simulink model "SIM_THREE_TANK_SERVO"  (R2025b)
settings: Solver=ode15s  StartTime=0.0  StopTime=1500  RelTol=1e-3
InitFcn:
  | run("index.m")
StopFcn:
  | data_name = "servo_response";
  | save_name = format_file_name(data_name,true);
  | 
  | % Save output data
  | save(save_name,"out")
values from neighbouring files (symbols this model uses):
  adaptParam = 0.15    [index.m]
  hiddenStates = 0    [index.m]
  model_const = struct()    [index.m]
undefined symbols (not defined in the file or in its folder): sigbuilder_block
libraries: simulink x1
settings Model: Creator=HP  LastModifiedBy=USER PC
settings RTWCC: GPUComputeCapability=3.5
settings GRTTargetCC: ArrayLayout=Row-major

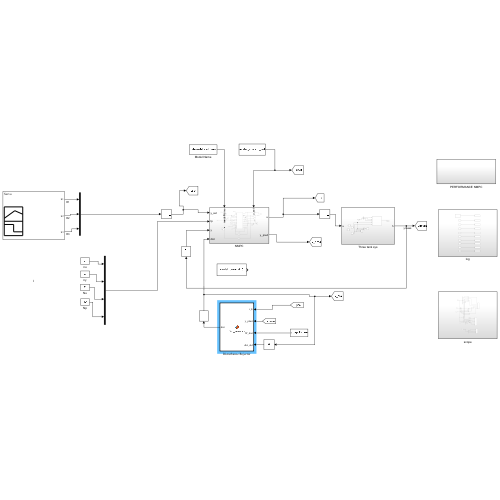
[thumbnail: Simulink's stored preview of the top-level diagram]
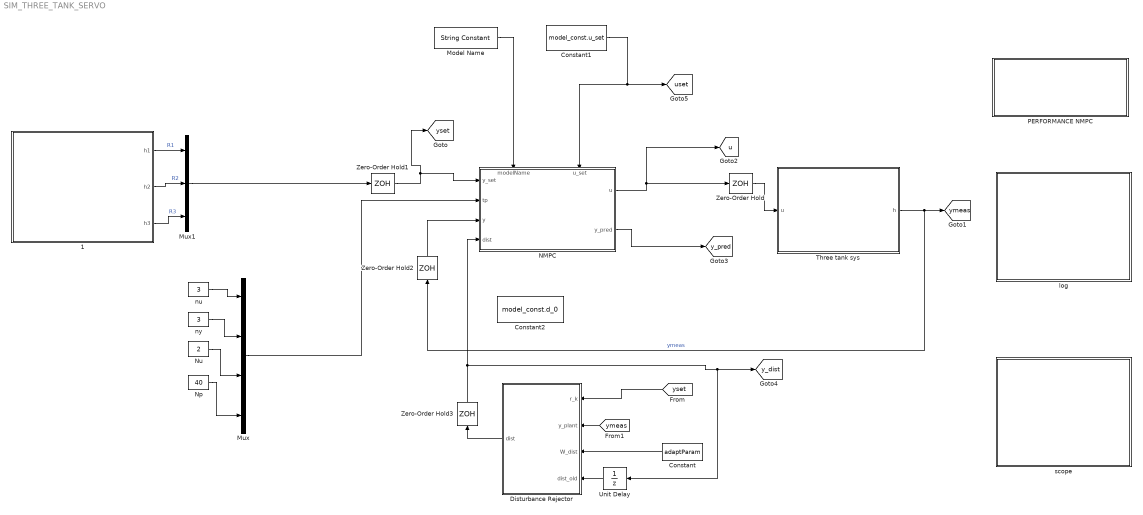
== system SIM_THREE_TANK_SERVO ==
  " 1" : Subsystem  Tag=STV Subsys  LoadFcn=sigbuilder_block('load');  StartFcn=sigbuilder_block('start');  StopFcn=sigbuilder_block('stop');  ClipboardFcn=sigbuilder_block('clipboard');  mask(Sigbuilder block){tuvar=[0:10]}
      mask help: Simulink:masks:SigbuilderBlock_MD
      mask init:
      | if ~strcmp(get_param(bdroot(gcbh),'SimulationStatus'),'stopped') tuvar = sigbuilder_block('maskInit'); end
      settings: CopyFcn=sigbuilder_block('copy');  DeleteFcn=sigbuilder_block('delete');  ModelCloseFcn=sigbuilder_block('modelClose');  PreSaveFcn=sigbuilder_block('preSave');  PauseFcn=sigbuilder_block('pause');  ContinueFcn=sigbuilder_block('continue');  NameChangeFcn=sigbuilder_block('namechange');  OpenFcn=sigbuilder_block('open',[316.5 171.75 805.5 485.25 ]);  CloseFcn=sigbuilder_block('close');
      mask Display: plot(0, 0, 100, 100,[2, 2, 32, 32, 2], [68, 8, 8, 68, 68],[32, 2], [38, 38], [32, 19, 2],[53, 60, 44], [32, 17, 17, 2],[16, 16, 31, 31]);txt = getActiveGroup(gcbh);text(2, 100, txt,'verticalAlignment', 'top');
  Constant : Constant  Value=adaptParam
  Constant1 : Constant  Value=model_const.u_set
  Constant2 : Constant  Value=model_const.d_0  SampleTime=model_const.ts
  Disturbance Rejector : MATLAB Function  TreatAsAtomicUnit=on  SystemSampleTime=10
  Model Name : StringConstant  String=networkModelName
  Mux : Mux
  Mux1 : Mux  Inputs=3
  NMPC : Subsystem
      settings: PortSchema="{\"entries\":[{\"content\":{\"sides\":[{\"content\":{\"connectorIds\":[\"In1\",\"In2\",\"In3\",\"In4\"]},\"type\":\"ConnectorPlacement.EquallySpacedRectSide\",\"uuid\":\"b907109f-bf70-45ef-b014-879f3ccfb12e\"},{\"content\":{\"connectorIds\":[\"Out1\",\"Out2\"],\"side\":\"RIGHT\"},\"type\":\"ConnectorPlacement.EquallySpacedRectSide\",\"uuid\":\"26d01547-fbc3-4b4e-b6e6-c22ae9e5b6d6\"},{\"content\":{\"connectorIds\":[\"In5\",\"In6\"],\"side\":\"TOP\"},\"type\":\"ConnectorPlacement.EquallySpacedRectSide\",\"uuid\":\"f1d5a2c8-1fb2-4706-a136-ec661fe312a9\"},{\"content\":{\"side\":\"BOTTOM\"},\"type\":\"ConnectorPlacement.EquallySpacedRectSide\",\"uuid\":\"24667040-ec86-4e57-b699-830e3f360007\"}]},\"type\":\"ConnectorPlacement.EquallySpacedConnector\",\"uuid\":\"8e79e654-12d3-4871-a9fc-130c68b7f74a\"}],\"packageUris\":[\"http://schema.mathworks.com/mf0/Connector/R2020b\"],\"version\":\"1.0\"}"
  Np : Constant  Value=40
  Nu : Constant  Value=2
  PERFORMANCE NMPC : Subsystem
  Three tank sys : Subsystem
  Unit Delay : UnitDelay  InitialCondition=model_const.d_0  SampleTime=model_const.ts  HasFrameUpgradeWarning=on
  Zero-Order Hold{,1..3} (4 alike) : ZeroOrderHold  SampleTime=model_const.ts
  log : Subsystem
  nu : Constant  Value=3
  ny : Constant  Value=3
  scope : Subsystem
  tag scope: u=global, uset=global, y_dist=global, y_pred=global, ymeas=global, yset=global
  wires:
  Zero-Order Hold1/1 -> NMPC/1(y_set), [yset]
  Nu/1 -> Mux/3
  Constant/1 -> Disturbance Rejector/3(W_dist)
  Unit Delay/1 -> Disturbance Rejector/4(dist_old)
  Mux/1 -> NMPC/2(tp)
  Np/1 -> Mux/4
  [ymeas] -> Disturbance Rejector/2(y_plant)
  NMPC/1(u) -> [u], Zero-Order Hold/1
  Model Name/1 -> NMPC/5(modelName)
  nu/1 -> Mux/1
  ny/1 -> Mux/2
  Constant1/1 -> NMPC/6(u_set), [uset]
  [yset] -> Disturbance Rejector/1(r_k)
  Zero-Order Hold3/1 -> NMPC/4(dist), Unit Delay/1, [y_dist]
  Zero-Order Hold/1 -> Three tank sys/1(u)
  NMPC/2(y_pred) -> [y_pred]
  Disturbance Rejector/1(dist) -> Zero-Order Hold3/1
  Three tank sys/1(h) -> Zero-Order Hold2/1, [ymeas]  "ymeas"
  Mux1/1 -> Zero-Order Hold1/1
  Zero-Order Hold2/1 -> NMPC/3(y)
  " 1"/3(h3) -> Mux1/3  "R3"
  " 1"/2(h2) -> Mux1/2  "R2"
  " 1"/1(h1) -> Mux1/1  "R1"

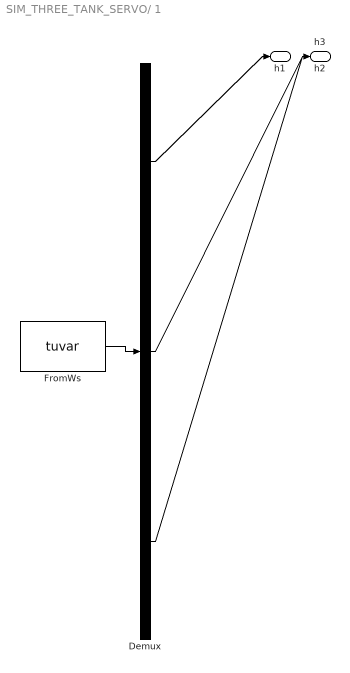
== system SIM_THREE_TANK_SERVO/ 1 ==
  Demux : Demux  Tag=STV Demux  Outputs=3
      settings: DisplayOption=none
  FromWs : FromWorkspace  Tag=STV FromWs  VariableName=tuvar  SampleTime=1
      SigBuilderData=|
      | common.afterFinalStr = 'Extrapolate'
      | common.sampleTime = '1'
      | dataSet.timeRange = [0 1500]
      | dataSet.name = 'Servo'
      | sbobj.Groups.Name = 'Servo'
      | sbobj.Groups.Signals(1).Name = 'h1'
      | sbobj.Groups.Signals(1).XData = [0 400 400 1500]
      | sbobj.Groups.Signals(1).YData = [14.29 14.29 20 20]
      | sbobj.Groups.Signals(2).Name = 'h2'
      | sbobj.Groups.Signals(2).XData = [0 800 800 1500]
      | sbobj.Groups.Signals(2).YData = [13.51 13.51 20 20]
      | sbobj.Groups.Signals(3).Name = 'h3'
      | sbobj.Groups.Signals(3).XData = [0 1200 1200 1500]
      | sbobj.Groups.Signals(3).YData = [16.06 16.06 20 20]
      | sbobj.Groups.TimeRange = [0 1500]
  h1 : Outport  Tag=STV Outport  VectorParamsAs1DForOutWhenUnconnected=off
  h2 : Outport  Tag=STV Outport  Port=2  VectorParamsAs1DForOutWhenUnconnected=off
  h3 : Outport  Tag=STV Outport  Port=3  VectorParamsAs1DForOutWhenUnconnected=off
  wires:
  FromWs/1 -> Demux/1
  Demux/1 -> h1/1
  Demux/2 -> h2/1
  Demux/3 -> h3/1

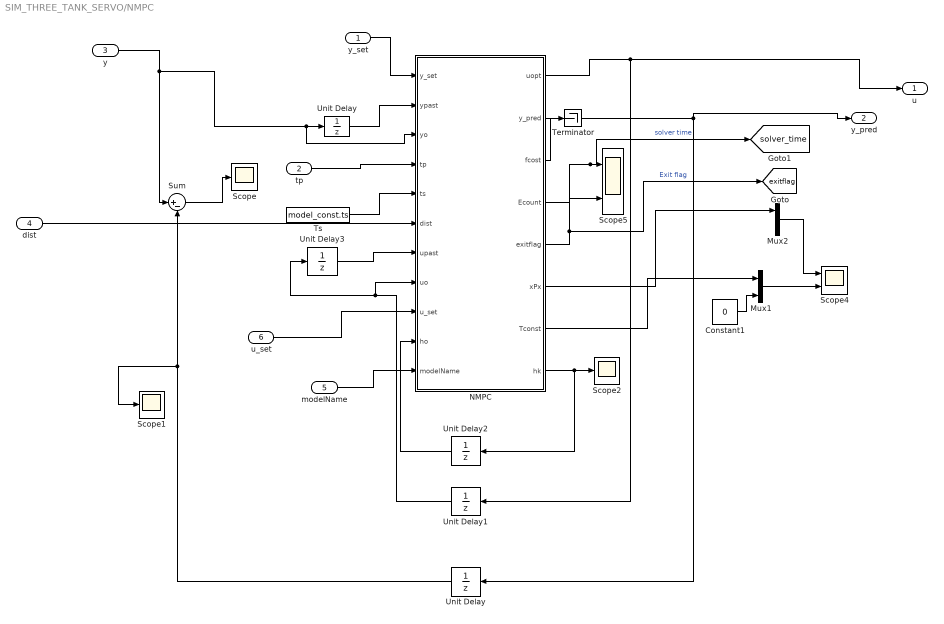
== system SIM_THREE_TANK_SERVO/NMPC ==
  y_set : Inport
  tp : Inport  Port=2
  y : Inport  Port=3
  dist : Inport  Port=4
  modelName : Inport  Port=5
  u_set : Inport  Port=6
  "  Unit Delay  " : UnitDelay  InitialCondition=model_const.y_0  SampleTime=model_const.ts  HasFrameUpgradeWarning=on
  " Unit Delay " : UnitDelay  InitialCondition=[0 0 0 ]  SampleTime=model_const.ts  HasFrameUpgradeWarning=on
  Constant1 : Constant  Value=0
  Mux1 : Mux  Inputs=2
  Mux2 : Mux  Inputs=2
  "NMPC " : MATLAB Function  TreatAsAtomicUnit=on  SystemSampleTime=model_const.ts
  Scope : Scope
      settings: ActiveDisplayYMinimum=-0.81983  ActiveDisplayYMaximum=1.85991
  Scope1 : Scope
      settings: ActiveDisplayYMinimum=2.45433  ActiveDisplayYMaximum=11.20291
  Scope2 : Scope
      settings: ActiveDisplayYMinimum=-0.0970614142715931  ActiveDisplayYMaximum=0.12913854792714119
  Scope4 : Scope  NumInputPorts=2
      settings: ActiveDisplayYMinimum=-0.25  ActiveDisplayYMaximum=2.25  DataLoggingVariableName=ScopeData2
  Scope5 : Scope  NumInputPorts=2
      settings: ShowGrid=off  ActiveDisplayYMinimum=1  ActiveDisplayYMaximum=3  DataLoggingVariableName=ScopeData3
  Sum : Sum  Inputs=|+-
  "Terminator " : Terminator
  Ts : Constant  Value=model_const.ts
  Unit Delay1 : UnitDelay  InitialCondition=model_const.u_0  SampleTime=model_const.ts  HasFrameUpgradeWarning=on
  Unit Delay2 : UnitDelay  InitialCondition=hiddenStates  SampleTime=model_const.ts  HasFrameUpgradeWarning=on
  Unit Delay3 : UnitDelay  InitialCondition=model_const.u_0  SampleTime=model_const.ts  HasFrameUpgradeWarning=on
  u : Outport  VectorParamsAs1DForOutWhenUnconnected=off
  y_pred : Outport  Port=2  VectorParamsAs1DForOutWhenUnconnected=off
  tag scope: exitflag=global, solver_time=global
  wires:
  y_set/1 -> "NMPC "/1(y_set)
  tp/1 -> "NMPC "/4(tp)
  Ts/1 -> "NMPC "/5(ts)
  "NMPC "/3(fcost) -> "Terminator "/1
  y/1 -> Sum/1, " Unit Delay "/1, "NMPC "/3(yo)
  "  Unit Delay  "/1 -> Scope1/1, Sum/2
  Sum/1 -> Scope/1
  dist/1 -> "NMPC "/6(dist)
  Constant1/1 -> Mux1/2
  Mux2/1 -> Scope4/1
  Mux1/1 -> Scope4/2
  "NMPC "/7(Tconst) -> Mux1/1
  "NMPC "/6(xPx) -> Mux2/1
  "NMPC "/4(Ecount) -> [solver_time], Scope5/1  "solver time"
  "NMPC "/5(exitflag) -> [exitflag], Scope5/2  "Exit flag"
  "NMPC "/8(hk) -> Unit Delay2/1, Scope2/1
  Unit Delay2/1 -> "NMPC "/10(ho)
  modelName/1 -> "NMPC "/11(modelName)
  "NMPC "/1(uopt) -> Unit Delay1/1, u/1
  Unit Delay1/1 -> Unit Delay3/1, "NMPC "/8(uo)
  " Unit Delay "/1 -> "NMPC "/2(ypast)
  Unit Delay3/1 -> "NMPC "/7(upast)
  u_set/1 -> "NMPC "/9(u_set)
  "NMPC "/2(y_pred) -> y_pred/1, "  Unit Delay  "/1

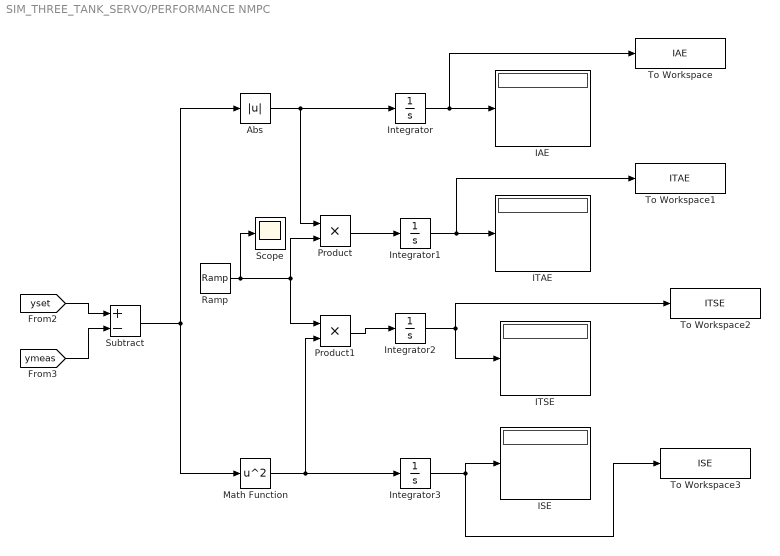
== system SIM_THREE_TANK_SERVO/PERFORMANCE NMPC ==
  Abs : Abs  SaturateOnIntegerOverflow=off
  IAE : Display
  ISE : Display
  ITAE : Display
  ITSE : Display
  Integrator{,1..3} (4 alike) : Integrator
  Math Function : Math  Operator=square  SignedPower=on
  Product : Product  RndMeth=Zero
  Product1 : Product  RndMeth=Zero
  Ramp : simulink/Sources/Ramp  slope=1  start=0  InitialOutput=0
  Scope : Scope
      settings: DataLoggingSaveFormat=Array
  Subtract : Sum  Inputs=+-
  To Workspace : ToWorkspace  VariableName=IAE  SaveFormat=Structure With Time  SampleTime=3
      settings: Decimation=4
  To Workspace1 : ToWorkspace  VariableName=ITAE  SaveFormat=Structure With Time  SampleTime=3
      settings: Decimation=4
  To Workspace2 : ToWorkspace  VariableName=ITSE  SaveFormat=Structure With Time  SampleTime=3
      settings: Decimation=4
  To Workspace3 : ToWorkspace  VariableName=ISE  SaveFormat=Structure With Time  SampleTime=3
      settings: Decimation=4
  wires:
  Integrator1/1 -> To Workspace1/1, ITAE/1
  Integrator3/1 -> ISE/1, To Workspace3/1
  Product/1 -> Integrator1/1
  Product1/1 -> Integrator2/1
  Math Function/1 -> Product1/2, Integrator3/1
  Ramp/1 -> Scope/1, Product1/1, Product/2
  Integrator/1 -> To Workspace/1, IAE/1
  Abs/1 -> Product/1, Integrator/1
  Subtract/1 -> Abs/1, Math Function/1
  [yset] -> Subtract/1
  [ymeas] -> Subtract/2
  Integrator2/1 -> ITSE/1, To Workspace2/1

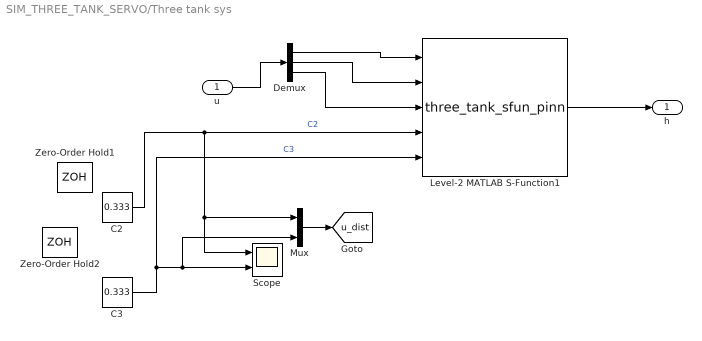
== system SIM_THREE_TANK_SERVO/Three tank sys ==
  u : Inport
  C2 : Constant  Value=0.333  SampleTime=model_const.ts
  C3 : Constant  Value=0.333  SampleTime=model_const.ts
  Demux : Demux  Outputs=3
  Level-2 MATLAB S-Function1 : M-S-Function  FunctionName=three_tank_sfun_pinn  Parameters=model_const.x_0
  Mux : Mux  Inputs=2
  Scope : Scope  NumInputPorts=2
      settings: Title=C3 valve opening  ShowGrid=off  ActiveDisplayYMinimum=0.239625  ActiveDisplayYMaximum=0.34337500000000004  DataLoggingVariableName=ScopeData5
  Zero-Order Hold1 : ZeroOrderHold  SampleTime=model_const.ts
  Zero-Order Hold2 : ZeroOrderHold  SampleTime=model_const.ts
  h : Outport
  tag scope: u_dist=global
  wires:
  Demux/2 -> Level-2 MATLAB S-Function1/2
  Level-2 MATLAB S-Function1/1 -> h/1
  u/1 -> Demux/1
  Demux/3 -> Level-2 MATLAB S-Function1/3
  Demux/1 -> Level-2 MATLAB S-Function1/1
  C3/1 -> Level-2 MATLAB S-Function1/5, Mux/2, Scope/2  "C3"
  C2/1 -> Scope/1, Mux/1, Level-2 MATLAB S-Function1/4  "C2"
  Mux/1 -> [u_dist]

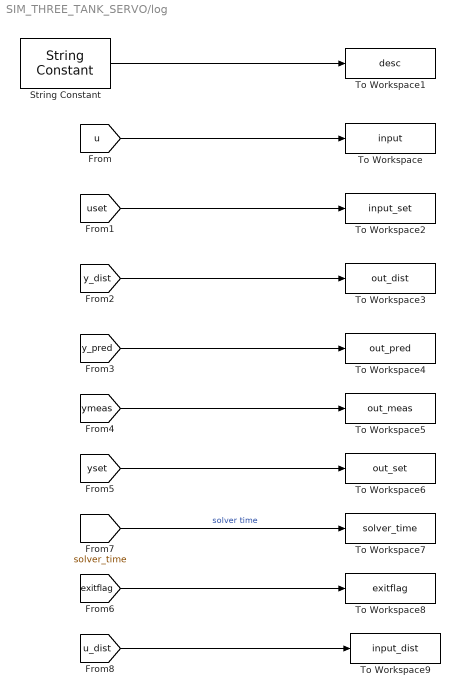
== system SIM_THREE_TANK_SERVO/log ==
  String Constant : StringConstant  String=description
  To Workspace : ToWorkspace  VariableName=input  SaveFormat=Structure With Time  SampleTime=model_const.ts
      settings: Decimation=2
  To Workspace1 : ToWorkspace  VariableName=desc  SaveFormat=Structure With Time  SampleTime=model_const.ts
      settings: Decimation=2
  To Workspace2 : ToWorkspace  VariableName=input_set  SaveFormat=Structure With Time  SampleTime=model_const.ts
      settings: Decimation=2
  To Workspace3 : ToWorkspace  VariableName=out_dist  SaveFormat=Structure With Time  SampleTime=model_const.ts
      settings: Decimation=2
  To Workspace4 : ToWorkspace  VariableName=out_pred  SaveFormat=Structure With Time  SampleTime=model_const.ts
      settings: Decimation=2
  To Workspace5 : ToWorkspace  VariableName=out_meas  SaveFormat=Structure With Time  SampleTime=model_const.ts
      settings: Decimation=2
  To Workspace6 : ToWorkspace  VariableName=out_set  SaveFormat=Structure With Time  SampleTime=model_const.ts
      settings: Decimation=2
  To Workspace7 : ToWorkspace  VariableName=solver_time  SaveFormat=Structure With Time  SampleTime=model_const.ts
  To Workspace8 : ToWorkspace  VariableName=exitflag  SaveFormat=Structure With Time  SampleTime=model_const.ts
  To Workspace9 : ToWorkspace  VariableName=input_dist  SaveFormat=Structure With Time  SampleTime=model_const.ts
  wires:
  [u] -> To Workspace/1
  [yset] -> To Workspace6/1
  [ymeas] -> To Workspace5/1
  [y_pred] -> To Workspace4/1
  [y_dist] -> To Workspace3/1
  [uset] -> To Workspace2/1
  String Constant/1 -> To Workspace1/1
  [solver_time] -> To Workspace7/1  "solver time"
  [exitflag] -> To Workspace8/1
  [u_dist] -> To Workspace9/1

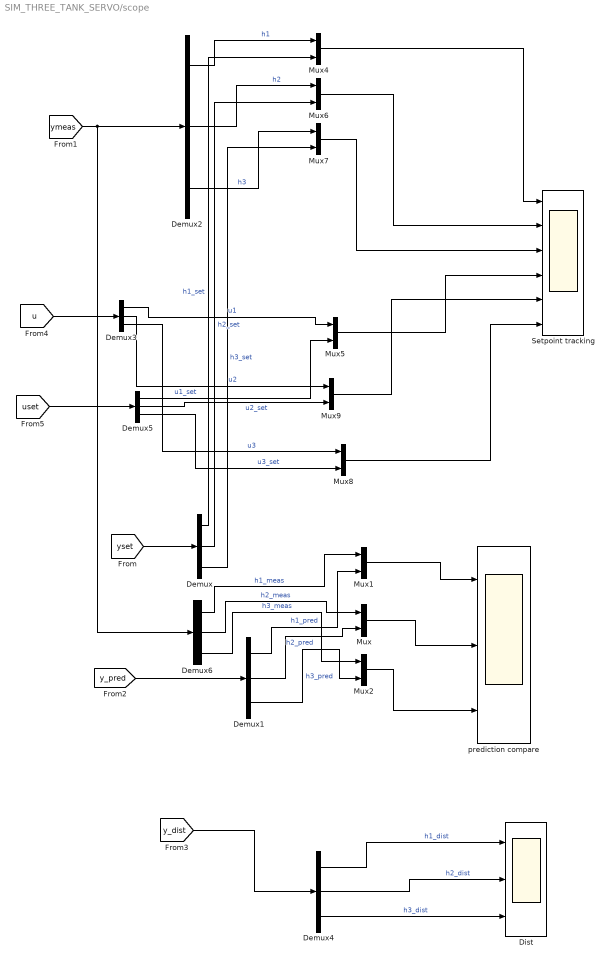
== system SIM_THREE_TANK_SERVO/scope ==
  Demux{,1..6} (7 alike) : Demux  Outputs=3
  Dist : Scope  NumInputPorts=3
      settings: ShowGrid=off  ActiveDisplayYMinimum=-1.2420793505961463  ActiveDisplayYMaximum=0.24676083719583586  DataLoggingVariableName=dist
  Mux{,1..2,4..9} (9 alike) : Mux  Inputs=2
  Setpoint tracking : Scope  NumInputPorts=6
      settings: ActiveDisplayString=5  ShowGrid=off  ActiveDisplayYMinimum=0.20223090917076997  ActiveDisplayYMaximum=0.57505564762598371  DataLoggingVariableName=servo
  prediction compare : Scope  NumInputPorts=3
      settings: ShowGrid=off  ActiveDisplayYMinimum=3.0846705781094617  ActiveDisplayYMaximum=22.23796479701485  DataLoggingVariableName=error
  wires:
  Demux/1 -> Mux4/2  "h1_set"
  Mux2/1 -> prediction compare/3
  Mux1/1 -> prediction compare/1
  [yset] -> Demux/1
  [y_pred] -> Demux1/1
  Demux1/1 -> Mux1/2  "h1_pred"
  Demux1/2 -> Mux/2  "h2_pred"
  Demux1/3 -> Mux2/2  "h3_pred"
  Demux/2 -> Mux6/2  "h2_set"
  Demux/3 -> Mux7/2  "h3_set"
  Mux/1 -> prediction compare/2
  [u] -> Demux3/1
  Demux3/1 -> Mux5/1  "u1"
  Demux3/2 -> Mux9/1  "u2"
  Mux7/1 -> Setpoint tracking/3
  Mux6/1 -> Setpoint tracking/2
  Mux4/1 -> Setpoint tracking/1
  Demux2/1 -> Mux4/1  "h1"
  Demux2/2 -> Mux6/1  "h2"
  Demux2/3 -> Mux7/1  "h3"
  [y_dist] -> Demux4/1
  Demux4/1 -> Dist/1  "h1_dist"
  Demux4/2 -> Dist/2  "h2_dist"
  Demux4/3 -> Dist/3  "h3_dist"
  [uset] -> Demux5/1
  Demux5/1 -> Mux5/2  "u1_set"
  Demux5/2 -> Mux9/2  "u2_set"
  Mux5/1 -> Setpoint tracking/4
  Demux6/1 -> Mux1/1  "h1_meas"
  Demux6/2 -> Mux/1  "h2_meas"
  Demux6/3 -> Mux2/1  "h3_meas"
  Mux9/1 -> Setpoint tracking/5
  Mux8/1 -> Setpoint tracking/6
  Demux3/3 -> Mux8/1  "u3"
  Demux5/3 -> Mux8/2  "u3_set"
  [ymeas] -> Demux6/1, Demux2/1

== matlab function SIM_THREE_TANK_SERVO/NMPC/NMPC  ==
  data: uopt output; y_pred output; fcost output size=[1,1]; Ecount output; exitflag output; xPx output; Tconst output; y_set input; ypast input; yo input; tp input; ts input; dist input; upast input; uo input; u_set input; ho input; hk output; modelName input
function [uopt, y_pred, fcost, Ecount, exitflag, xPx, Tconst, hk] = nmpc(y_set, ypast, yo, tp, ts, dist, upast, uo, u_set, ho, modelName)
uopt = [0;0;0];
fcost = 0;
y_pred = [0;0;0];
% Regression
u_reg = [upast(1) upast(2), upast(3);uo(1) uo(2),uo(3)];
y_reg =[ypast';yo'];
Ecount = 0 ;
exitflag = Inf ;
xPx = 0 ;
Tconst = 0 ;
hk = ho;
% Steady states
h1ss=y_set(1) ; h2ss=y_set(2) ; h3ss=y_set(3) ;
u1ss=u_set(1) ; u2ss=u_set(2) ; u3ss = u_set(3);
rhox = 20;
rhou=10;
Wy = [1/h1ss, 1/h2ss, 1/h3ss]*rhox;
% FIX 1: no penalty on (u - u_set). u_set is a fixed nominal point and does
% not move with the setpoints, so penalising it dragged u1 toward 100 and
% forced the disturbance integrator to wind up. Wdu keeps the moves smooth.
Wu    = [0, 0, 0];
Wdu   = [1/u1ss,10/u2ss, 10/u3ss]*rhou;
Wuerr = [0, 0, 0];
P1 =[
    0.3408    0.1556    0.0754;
    0.1556    0.4888    0.2504;
    0.0754    0.2504    0.6810;];
alpha1 = 20.4206;
P=P1;
alpha = alpha1*rhox;
nu = tp(1);
ny = tp(2);
Nu = tp(3);
Np = tp(4);
bounds = struct();
bounds.ymin =[0.1 ,0.1, 0.1];
bounds.ymax =[35 35 35];
% FIX 2: input bounds = PINN training range (x_lo/x_hi in pinn_weights.mat),
% so the optimiser never asks the network to extrapolate.
bounds.u_min = [55,  0.17, 0.11];
bounds.u_max = [148, 1.00, 0.87];
du = [10, 0.1, 0.1];
bounds.du_min =  -du;
bounds.du_max = du;
params = struct();
params.y_set = y_set;
params.u_set = u_set;
params.nu = nu;
params.ny = ny;
params.Nu = Nu;
params.Np = Np;
params.Wy = Wy;
params.Wdu = Wdu;
params.Wu = Wu;
params.Wuerr =Wuerr;
params.ts = ts;
params.P = P;
params.alpha = alpha;
params.modelName = modelName;
params.bounds = bounds;
params.dist = dist;
coder.extrinsic('get_control_input');
[uopt, y_pred, hk, fval, exitflag, elapsed, ~, ~] = get_control_input(y_reg, u_reg, ho, params);
% FIX 3: get_control_input returns PINN + dist. The scope should show the
% raw PINN prediction, so remove the disturbance term here. y_pred only
% feeds the scope; the controller is unaffected.
y_pred = y_pred(:) - dist(:);
fcost = fval;
Ecount = elapsed ;
end

== matlab function SIM_THREE_TANK_SERVO/Disturbance Rejector ==
  data: r_k input; dist output; y_plant input; W_dist input; dist_old input
function dist = Dist_rejector(r_k, y_plant, W_dist, dist_old)
% DIST_REJECTOR: integral-type disturbance estimate for offset-free NMPC
%   dist_k = dist_{k-1} + W_dist * (y_k - r_k)
%
% Changes from the original:
%   1. Linear error instead of tanh(e). tanh saturated at |e| > ~2 cm, which
%      capped the update at W_dist per step and made large disturbances
%      recover along a slow straight line.
%   2. Anti-windup: integration is frozen for FREEZE_STEPS samples after any
%      setpoint change, so servo steps (large but expected tracking error)
%      do not wind the estimate up.
%   3. Estimate clamped to +/- D_MAX.
%
% Inputs:
%   r_k      - setpoint [3x1]
%   y_plant  - measured levels [3x1]
%   W_dist   - integration gain (scalar or [3x1])
%   dist_old - previous estimate [3x1]

FREEZE_STEPS = 30;   % 30 samples = 60 s at Ts = 2 s
D_MAX        = 15;   % cm

persistent r_prev hold_cnt
if isempty(r_prev)
    r_prev   = r_k;
    hold_cnt = 0;
end

% setpoint changed -> start freeze
if any(abs(r_k(:) - r_prev(:)) > 1e-6)
    hold_cnt = FREEZE_STEPS;
end
r_prev = r_k;

e_k = y_plant - r_k;

if hold_cnt > 0
    hold_cnt = hold_cnt - 1;
    dist = dist_old;                    % frozen
else
    dist = dist_old + W_dist .* e_k;    % linear integral update
end

dist = min(max(dist, -D_MAX), D_MAX);
end


% function dist = Dist_rejector(r_k, y_plant, W_dist, dist_old)
% % DIST_REJECTOR: Estimates disturbance based on output error
% %
% % Inputs:
% %   r_k      - Reference/predicted output (scalar or array)
% %   y_plant  - Actual plant output (scalar or array)
% %   W_dist   - Disturbance gain (scalar or array)
% %   dist_old - Previous disturbance estimate (scalar or array)
% %
% % Output:
% %   dist     - Updated disturbance estimate (same size as r_k)
%     % Compute element-wise error
%     % disp(size(r_k))
%     %   disp(size(y_plant))
%     %   disp(size(dist_old))
%     e_k = y_plant - r_k;
% 
%     % Permissible error bounds (change if needed)
%     error_min = -Inf;
%     error_max =  Inf;
% 
%     % Apply tanh only within bounds
%     valid_mask = (e_k > error_min) & (e_k < error_max);
%     error_func = zeros(size(e_k), 'like', e_k);
%     error_func(valid_mask) = tanh(e_k(valid_mask));
%     % Alternative: error_func(valid_mask) = e_k(valid_mask);
% 
%     % Element-wise disturbance update
%     dist = error_func .* W_dist + dist_old;
% end
